simulink model "Partie3_Detecteur"  (R2026b)
settings: Solver=FixedStepDiscrete  StopTime=1e7  FixedStep=Te
undefined symbols (not defined in the file): A, graine, graine_bruit, L, nErrMax, p1, Tb, Te, variance_bruit
libraries: simulink x1
settings Model: Creator=e2404931  LastModifiedBy=WORLD COMPUTERS
settings DataIOCC: ReturnWorkspaceOutputs=off

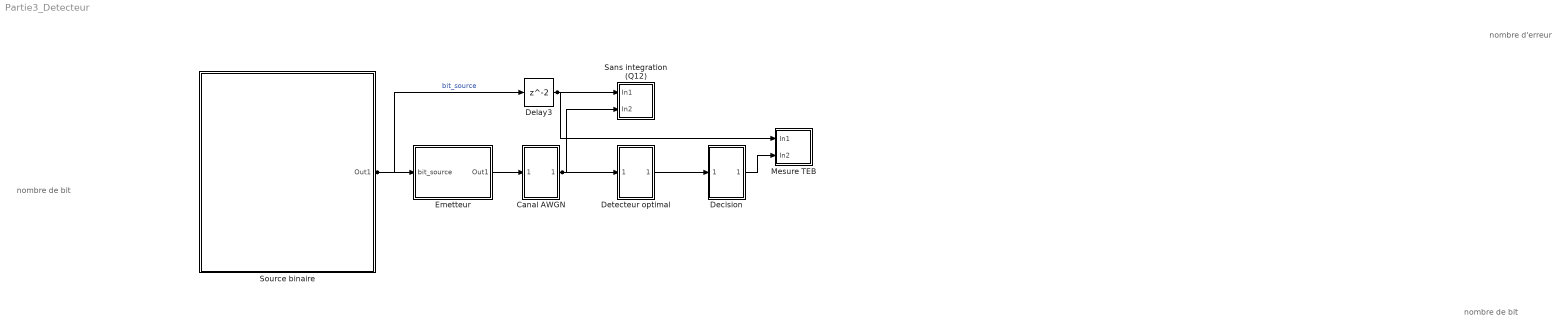
== system Partie3_Detecteur ==
  note: nombre d'erreur
  note: nombre de bit
  note: nombre de bit
  Canal AWGN : Subsystem
  Decision : Subsystem
  Delay3 : Delay
  Detecteur optimal : Subsystem
  Emetteur : Subsystem
  Mesure TEB : Subsystem
  Sans integration (Q12) : Subsystem
  Source binaire : Subsystem
  wires:
  Source binaire/1(Out1) -> Delay3/1, Emetteur/1(bit_source)  "bit_source"
  Detecteur optimal/1(Out1) -> Decision/1(In1)
  Emetteur/1(Out1) -> Canal AWGN/1(In1)
  Delay3/1 -> Mesure TEB/1(In1), Sans integration (Q12)/1(In1)
  Decision/1(Out1) -> Mesure TEB/2(In2)
  Canal AWGN/1(Out1) -> Detecteur optimal/1(In1), Sans integration (Q12)/2(In2)

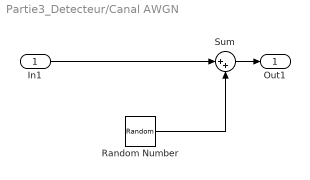
== system Partie3_Detecteur/Canal AWGN ==
  In1 : Inport
  Random Number : RandomNumber  Variance=variance_bruit  Seed=graine_bruit  SampleTime=Te
  Sum : Sum  Inputs=|++
  Out1 : Outport
  wires:
  Random Number/1 -> Sum/2
  Sum/1 -> Out1/1
  In1/1 -> Sum/1

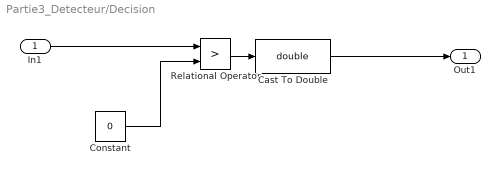
== system Partie3_Detecteur/Decision ==
  In1 : Inport
  Cast To Double : DataTypeConversion  OutDataTypeStr=double  SaturateOnIntegerOverflow=off  RndMeth=Floor
  Constant : Constant  Value=0
  Relational Operator : RelationalOperator  Operator=>  OutDataTypeStr=boolean  RndMeth=Simplest  InputSameDT=off
  Out1 : Outport
  wires:
  Relational Operator/1 -> Cast To Double/1
  Constant/1 -> Relational Operator/2
  In1/1 -> Relational Operator/1
  Cast To Double/1 -> Out1/1

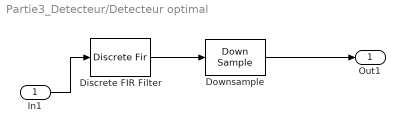
== system Partie3_Detecteur/Detecteur optimal ==
  In1 : Inport
  Discrete FIR Filter : DiscreteFir  Coefficients=ones(1,L)/L  OutDataTypeStr=Inherit: Same as accumulator
  Downsample : DownSample  DownsamplingFactor=L  SampleOffset=L-1  RateOptions=Allow multirate processing
  Out1 : Outport
  wires:
  Downsample/1 -> Out1/1
  In1/1 -> Discrete FIR Filter/1
  Discrete FIR Filter/1 -> Downsample/1

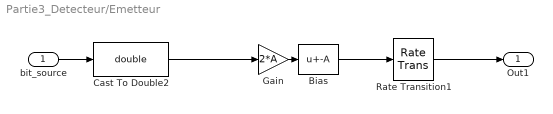
== system Partie3_Detecteur/Emetteur ==
  bit_source : Inport
  Bias : Bias  Bias=-A  SaturateOnIntegerOverflow=off
  Cast To Double2 : DataTypeConversion  OutDataTypeStr=double  SaturateOnIntegerOverflow=off  RndMeth=Floor
  Gain : Gain  Gain=2*A
  Rate Transition1 : RateTransition  InitialCondition=Tb  OutPortSampleTime=Te
  Out1 : Outport
  wires:
  Cast To Double2/1 -> Gain/1
  Bias/1 -> Rate Transition1/1
  bit_source/1 -> Cast To Double2/1
  Gain/1 -> Bias/1
  Rate Transition1/1 -> Out1/1

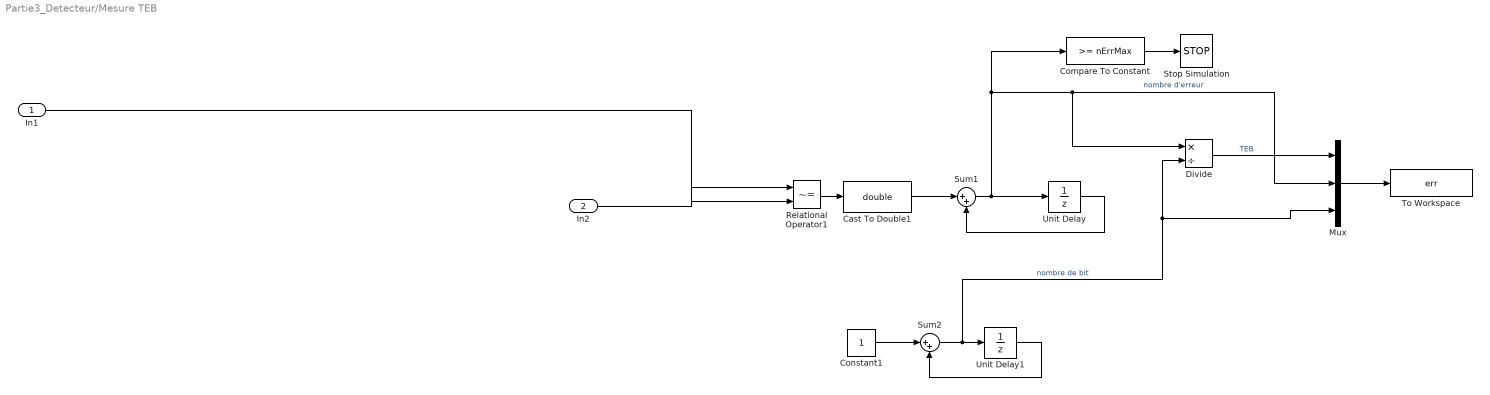
== system Partie3_Detecteur/Mesure TEB ==
  In1 : Inport
  In2 : Inport  Port=2
  Cast To Double1 : DataTypeConversion  OutDataTypeStr=double  SaturateOnIntegerOverflow=off  RndMeth=Floor
  Compare To Constant : simulink/Logic and Bit Operations/Compare To Constant  relop=>=  const=nErrMax  OutDataTypeStr=boolean
  Constant1 : Constant
  Divide : Product  Inputs=*/
  Mux : Mux  Inputs=3
  Relational Operator1 : RelationalOperator  Operator=~=  OutDataTypeStr=boolean  RndMeth=Simplest  InputSameDT=off
  Stop Simulation : Stop
  Sum1 : Sum  Inputs=|++
  Sum2 : Sum  Inputs=|++
  To Workspace : ToWorkspace  VariableName=err  SampleTime=-1
  Unit Delay : UnitDelay  SampleTime=Tb
  Unit Delay1 : UnitDelay  SampleTime=Tb
  wires:
  Compare To Constant/1 -> Stop Simulation/1
  Unit Delay/1 -> Sum1/2
  Sum1/1 -> Mux/2, Divide/1, Compare To Constant/1, Unit Delay/1  "nombre d'erreur"
  Constant1/1 -> Sum2/1
  Divide/1 -> Mux/1  "TEB"
  Relational Operator1/1 -> Cast To Double1/1
  Mux/1 -> To Workspace/1
  Cast To Double1/1 -> Sum1/1
  Unit Delay1/1 -> Sum2/2
  Sum2/1 -> Divide/2, Mux/3, Unit Delay1/1  "nombre de bit"
  In1/1 -> Relational Operator1/2
  In2/1 -> Relational Operator1/1

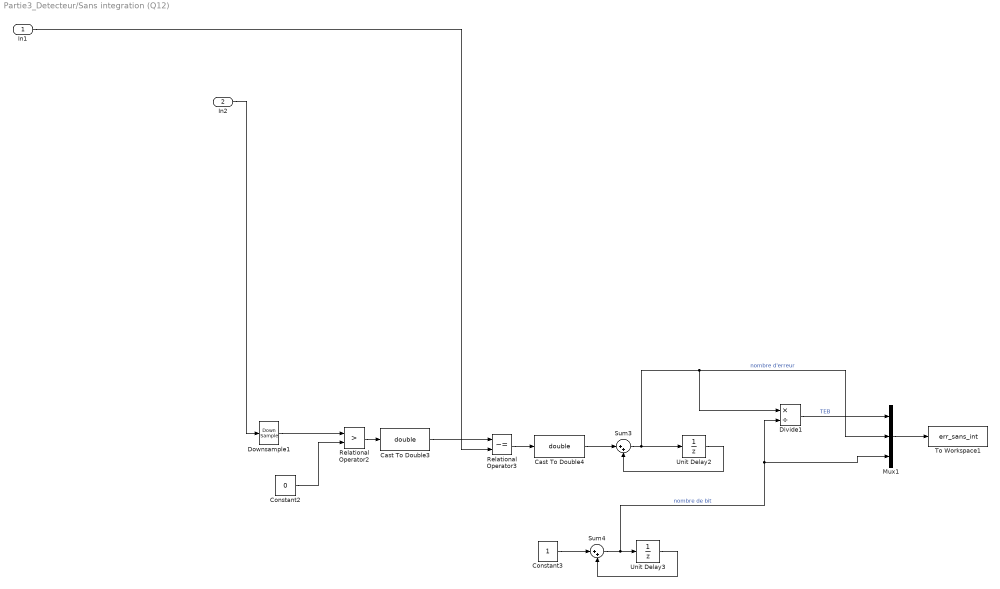
== system Partie3_Detecteur/Sans integration (Q12) ==
  In1 : Inport
  In2 : Inport  Port=2
  Cast To Double3 : DataTypeConversion  OutDataTypeStr=double  SaturateOnIntegerOverflow=off  RndMeth=Floor
  Cast To Double4 : DataTypeConversion  OutDataTypeStr=double  SaturateOnIntegerOverflow=off  RndMeth=Floor
  Constant2 : Constant  Value=0
  Constant3 : Constant
  Divide1 : Product  Inputs=*/
  Downsample1 : DownSample  DownsamplingFactor=L  SampleOffset=ech_milieu  RateOptions=Allow multirate processing
  Mux1 : Mux  Inputs=3
  Relational Operator2 : RelationalOperator  Operator=>  OutDataTypeStr=boolean  RndMeth=Simplest  InputSameDT=off
  Relational Operator3 : RelationalOperator  Operator=~=  OutDataTypeStr=boolean  RndMeth=Simplest  InputSameDT=off
  Sum3 : Sum  Inputs=|++
  Sum4 : Sum  Inputs=|++
  To Workspace1 : ToWorkspace  VariableName=err_sans_int  SampleTime=-1
  Unit Delay2 : UnitDelay  SampleTime=Tb
  Unit Delay3 : UnitDelay  SampleTime=Tb
  wires:
  In2/1 -> Downsample1/1
  Sum3/1 -> Mux1/2, Divide1/1, Unit Delay2/1  "nombre d'erreur"
  Cast To Double4/1 -> Sum3/1
  Divide1/1 -> Mux1/1  "TEB"
  Relational Operator2/1 -> Cast To Double3/1
  Cast To Double3/1 -> Relational Operator3/1
  Relational Operator3/1 -> Cast To Double4/1
  Downsample1/1 -> Relational Operator2/1
  Mux1/1 -> To Workspace1/1
  Unit Delay2/1 -> Sum3/2
  Sum4/1 -> Divide1/2, Mux1/3, Unit Delay3/1  "nombre de bit"
  Constant2/1 -> Relational Operator2/2
  Constant3/1 -> Sum4/1
  Unit Delay3/1 -> Sum4/2
  In1/1 -> Relational Operator3/2

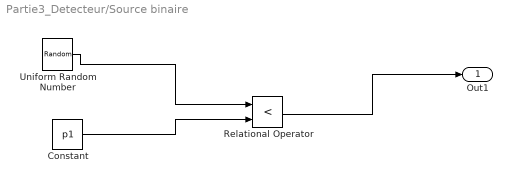
== system Partie3_Detecteur/Source binaire ==
  Constant : Constant  Value=p1
  Relational Operator : RelationalOperator  Operator=<  OutDataTypeStr=boolean  RndMeth=Simplest  InputSameDT=off
  Uniform Random Number : UniformRandomNumber  Minimum=0  Seed=graine  SampleTime=Tb
  Out1 : Outport
  wires:
  Uniform Random Number/1 -> Relational Operator/1
  Constant/1 -> Relational Operator/2
  Relational Operator/1 -> Out1/1
